simulink model "EFB"  (R2022b)
settings: Solver=FixedStepDiscrete  StartTime=0.0  StopTime=0.01  RelTol=1e-3
libraries: dspsrcs4 x1
settings Model: Creator=ASAA  LastModifiedBy=ASAA

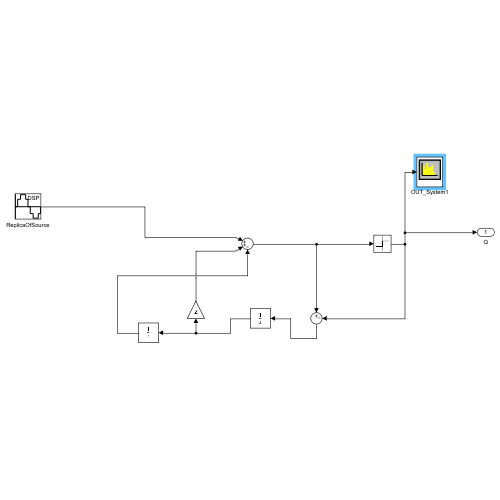
[thumbnail: Simulink's stored preview of the top-level diagram]
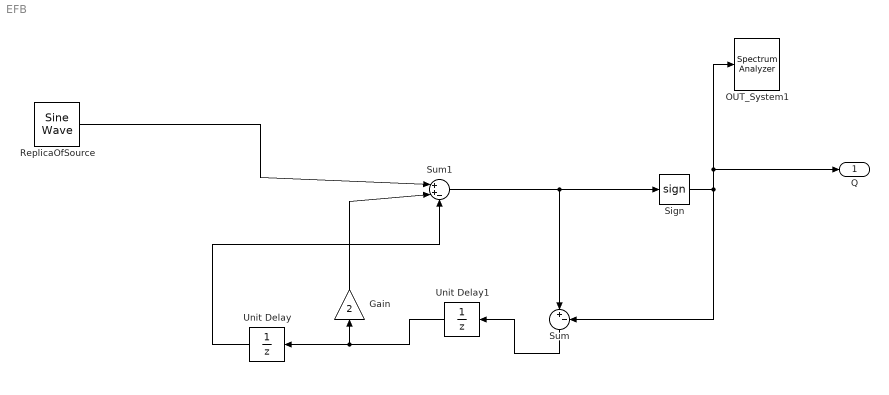
== system EFB ==
  Gain : Gain  Gain=2  OutDataTypeStr=fixdt(1,16,12)  SaturateOnIntegerOverflow=on
  OUT_System1 : SpectrumAnalyzer
  ReplicaOfSource : dspsrcs4/Sine Wave  Amplitude=0.6  Frequency=100e3  Phase=0  SampleMode=Discrete  OutComplex=Real  CompMethod=Trigonometric fcn  TableSize=Speed  SampleTime=1/3.125e6  SamplesPerFrame=1  ResetState=Restart at time zero  OutputFrames=off  dataType=double  wordLen=16  udDataType=sfix(16)  fracBitsMode=Best precision  numFracBits=15  OutDataTypeStr=double  LastOutDataTypeStr=double
  Sign : Signum
  Sum : Sum  Inputs=|+-  OutDataTypeStr=fixdt(1,16,13)  RndMeth=Nearest  SaturateOnIntegerOverflow=on
  Sum1 : Sum  Inputs=|++-  OutDataTypeStr=fixdt(1,16,12)  SaturateOnIntegerOverflow=on
  Unit Delay : UnitDelay  SampleTime=1e-8  HasFrameUpgradeWarning=on
  Unit Delay1 : UnitDelay  SampleTime=1e-8  HasFrameUpgradeWarning=on
  Q : Outport
  wires:
  Unit Delay1/1 -> Unit Delay/1, Gain/1
  Unit Delay/1 -> Sum1/3
  Sum/1 -> Unit Delay1/1
  Sum1/1 -> Sign/1, Sum/1
  Gain/1 -> Sum1/2
  Sign/1 -> Q/1, OUT_System1/1, Sum/2
  ReplicaOfSource/1 -> Sum1/1
